simulink model "Chen2003_ExtendedEMF"  (R2024b)
settings: Solver=FixedStepDiscrete  StartTime=0.0  StopTime=.52  FixedStep=Ts  RelTol=1e-3
model workspace (MAT data in the model file):
  Bobs = 850
  ID0 = -2
  IQ0 = 2
  KiPLL = 5600
  KpPLL = 150
  Ld = 0.00159999995958
  Lq = 0.00310000008903
  Omega0 = 280
  PolePairs = 4
  PsiPM = 0.0450000017881
  RecordedSignalNames = {'VAlpha'; 'VBeta'; 'IAlpha'; 'IBeta'; 'ThetaTrue'; 'ID'; 'IQ'; 'Torque'; 'BaselineTheta'; 'BaselineOmega'; 'BaselineEAlpha'; 'BaselineEBeta'; 'EEMFTheta'; 'EEMFOmega'; 'EEMFEAlpha'; 'EEMFEBeta'}
  Rs = 0.20000000298
  ScenarioInput = timeseries
  ScenarioInput.Name = 'unnamed'
  ScenarioInput.DataInfo = tsdata.datametadata
  ScenarioInput.DataInfo.Interpolation = tsdata.interpolation
  ScenarioInput.DataInfo.Interpolation.Fhandle : function handle (value not decoded)
  ScenarioInput.DataInfo.Interpolation.Name = 'linear'
  ScenarioInput.TimeInfo = tsdata.timemetadata
  ScenarioInput.TimeInfo.Length = 10401
  ScenarioInput.TimeInfo.DuplicateTimes = 0
  ScenarioInput.TimeInfo.Time_ = [0 5e-05 0.0001 0.00015 0.0002 0.00025 0.0003 0.00035 0.0004 0.00045 0.0005 0.00055 ... (10401 elements, 10401x1)]
  ScenarioInput.TimeInfo.Initialized = 1
  ScenarioInput.QualityInfo = tsdata.qualmetadata
  ScenarioInput.Data_ = [-7.32373666763 -7.5133357048 -7.70101070404 -7.88671445847 -8.07039928436 -8.25201797485 -8.43152427673 -8.60887241364 -8.78401660919 -8.95691204071 -9.12751483917 -9.29578113556 ... (41604 elements, 10401x4)]
  Theta0 = 0.119999997318
  ThetaPlant = 0.379999995232
  Ts = 5e-05
  Vdc = 60
settings Model: Creator=lxy  LastModifiedBy=lxy

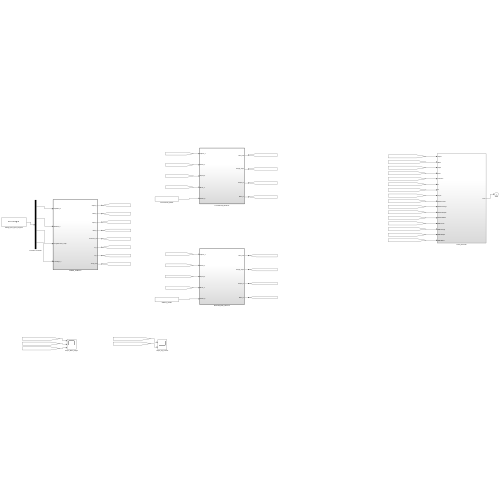
[thumbnail: Simulink's stored preview of the top-level diagram]
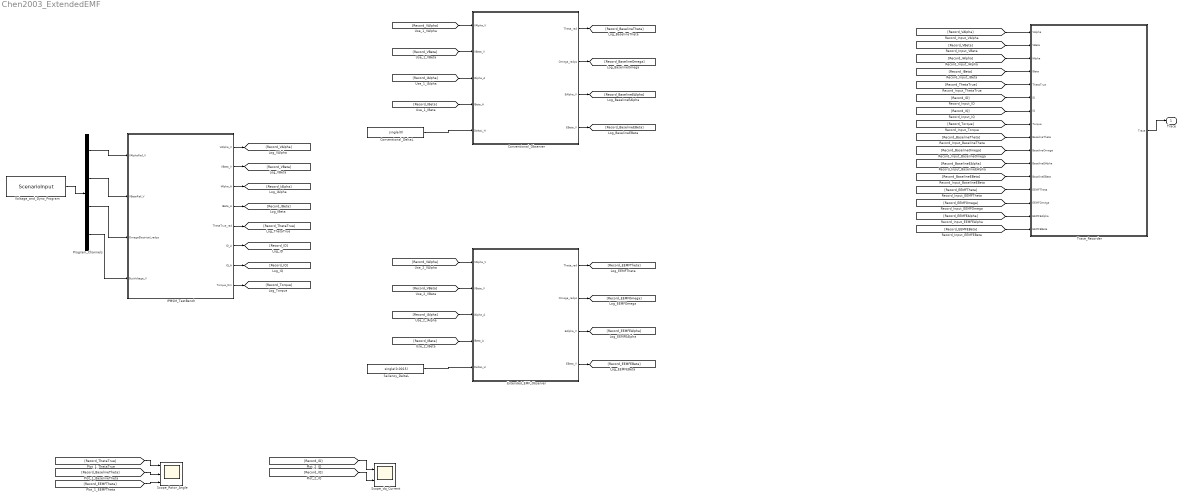
== system Chen2003_ExtendedEMF ==
  Conventional_DeltaL : Constant  Value=single(0)
  Conventional_Observer : Subsystem  TreatAsAtomicUnit=on
  Extended_EMF_Observer : Subsystem  TreatAsAtomicUnit=on
  IPMSM_TestBench : Subsystem  TreatAsAtomicUnit=on
  Program_Channels : Demux
  Saliency_DeltaL : Constant  Value=single(0.0015)
  Scope_Rotor_Angle : Scope  NumInputPorts=3
  Scope_dq_Current : Scope  NumInputPorts=2
  Trace_Recorder : Subsystem
  Voltage_and_Dyno_Program : FromWorkspace  VariableName=ScenarioInput  SampleTime=Ts  Interpolate=off  OutputAfterFinalValue=Holding final value
  Trace : Outport
  wires:
  Program_Channels/4 -> IPMSM_TestBench/4(BusVoltage_V)
  Program_Channels/2 -> IPMSM_TestBench/2(VBetaRef_V)
  Program_Channels/1 -> IPMSM_TestBench/1(VAlphaRef_V)
  Program_Channels/3 -> IPMSM_TestBench/3(OmegaElectrical_radps)
  Voltage_and_Dyno_Program/1 -> Program_Channels/1
  Saliency_DeltaL/1 -> Extended_EMF_Observer/5(DeltaL_H)
  Conventional_DeltaL/1 -> Conventional_Observer/5(DeltaL_H)
  [Record_EEMFEBeta] -> Trace_Recorder/16(EEMFEBeta)
  [Record_EEMFEAlpha] -> Trace_Recorder/15(EEMFEAlpha)
  [Record_EEMFOmega] -> Trace_Recorder/14(EEMFOmega)
  [Record_EEMFTheta] -> Trace_Recorder/13(EEMFTheta)
  [Record_BaselineEBeta] -> Trace_Recorder/12(BaselineEBeta)
  [Record_BaselineEAlpha] -> Trace_Recorder/11(BaselineEAlpha)
  [Record_BaselineOmega] -> Trace_Recorder/10(BaselineOmega)
  [Record_BaselineTheta] -> Trace_Recorder/9(BaselineTheta)
  [Record_Torque] -> Trace_Recorder/8(Torque)
  [Record_IQ] -> Trace_Recorder/7(IQ)
  [Record_ID] -> Trace_Recorder/6(ID)
  [Record_ThetaTrue] -> Trace_Recorder/5(ThetaTrue)
  [Record_IBeta] -> Trace_Recorder/4(IBeta)
  [Record_IAlpha] -> Trace_Recorder/3(IAlpha)
  [Record_VBeta] -> Trace_Recorder/2(VBeta)
  [Record_VAlpha] -> Trace_Recorder/1(VAlpha)
  Trace_Recorder/1(Trace) -> Trace/1
  Extended_EMF_Observer/4(EBeta_V) -> [Record_EEMFEBeta]
  Extended_EMF_Observer/3(EAlpha_V) -> [Record_EEMFEAlpha]
  Extended_EMF_Observer/2(Omega_radps) -> [Record_EEMFOmega]
  Conventional_Observer/4(EBeta_V) -> [Record_BaselineEBeta]
  Conventional_Observer/3(EAlpha_V) -> [Record_BaselineEAlpha]
  Conventional_Observer/2(Omega_radps) -> [Record_BaselineOmega]
  IPMSM_TestBench/8(Torque_Nm) -> [Record_Torque]
  Extended_EMF_Observer/1(Theta_rad) -> [Record_EEMFTheta]
  Conventional_Observer/1(Theta_rad) -> [Record_BaselineTheta]
  IPMSM_TestBench/5(ThetaTrue_rad) -> [Record_ThetaTrue]
  IPMSM_TestBench/2(VBeta_V) -> [Record_VBeta]
  IPMSM_TestBench/1(VAlpha_V) -> [Record_VAlpha]
  IPMSM_TestBench/3(IAlpha_A) -> [Record_IAlpha]
  IPMSM_TestBench/4(IBeta_A) -> [Record_IBeta]
  IPMSM_TestBench/6(ID_A) -> [Record_ID]
  IPMSM_TestBench/7(IQ_A) -> [Record_IQ]
  [Record_IBeta] -> Extended_EMF_Observer/4(IBeta_A)
  [Record_IAlpha] -> Extended_EMF_Observer/3(IAlpha_A)
  [Record_VBeta] -> Extended_EMF_Observer/2(VBeta_V)
  [Record_VAlpha] -> Extended_EMF_Observer/1(VAlpha_V)
  [Record_IBeta] -> Conventional_Observer/4(IBeta_A)
  [Record_IAlpha] -> Conventional_Observer/3(IAlpha_A)
  [Record_VBeta] -> Conventional_Observer/2(VBeta_V)
  [Record_VAlpha] -> Conventional_Observer/1(VAlpha_V)
  [Record_IQ] -> Scope_dq_Current/2
  [Record_ID] -> Scope_dq_Current/1
  [Record_EEMFTheta] -> Scope_Rotor_Angle/3
  [Record_BaselineTheta] -> Scope_Rotor_Angle/2
  [Record_ThetaTrue] -> Scope_Rotor_Angle/1

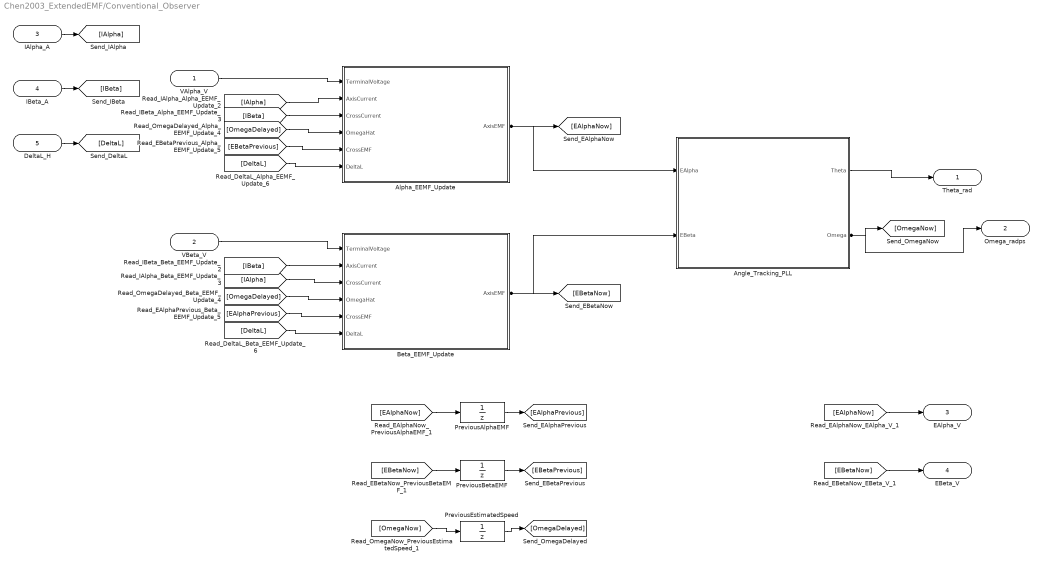
== system Chen2003_ExtendedEMF/Conventional_Observer ==
  VAlpha_V : Inport  OutDataTypeStr=single  SampleTime=Ts
  VBeta_V : Inport  Port=2  OutDataTypeStr=single  SampleTime=Ts
  IAlpha_A : Inport  Port=3  OutDataTypeStr=single  SampleTime=Ts
  IBeta_A : Inport  Port=4  OutDataTypeStr=single  SampleTime=Ts
  DeltaL_H : Inport  Port=5  OutDataTypeStr=single  SampleTime=Ts
  Alpha_EEMF_Update : Subsystem
  Angle_Tracking_PLL : Subsystem
  Beta_EEMF_Update : Subsystem
  PreviousAlphaEMF : UnitDelay  SampleTime=Ts  HasFrameUpgradeWarning=on
  PreviousBetaEMF : UnitDelay  SampleTime=Ts  HasFrameUpgradeWarning=on
  PreviousEstimatedSpeed : UnitDelay  InitialCondition=Omega0  SampleTime=Ts  HasFrameUpgradeWarning=on
  Theta_rad : Outport
  Omega_radps : Outport  Port=2
  EAlpha_V : Outport  Port=3
  EBeta_V : Outport  Port=4
  wires:
  [OmegaDelayed] -> Beta_EEMF_Update/4(OmegaHat)
  [OmegaDelayed] -> Alpha_EEMF_Update/4(OmegaHat)
  PreviousEstimatedSpeed/1 -> [OmegaDelayed]
  [OmegaNow] -> PreviousEstimatedSpeed/1
  [EBetaPrevious] -> Alpha_EEMF_Update/5(CrossEMF)
  PreviousBetaEMF/1 -> [EBetaPrevious]
  [EBetaNow] -> EBeta_V/1
  [EBetaNow] -> PreviousBetaEMF/1
  [EAlphaPrevious] -> Beta_EEMF_Update/5(CrossEMF)
  PreviousAlphaEMF/1 -> [EAlphaPrevious]
  [EAlphaNow] -> EAlpha_V/1
  [EAlphaNow] -> PreviousAlphaEMF/1
  [DeltaL] -> Beta_EEMF_Update/6(DeltaL)
  [DeltaL] -> Alpha_EEMF_Update/6(DeltaL)
  DeltaL_H/1 -> [DeltaL]
  [IBeta] -> Beta_EEMF_Update/2(AxisCurrent)
  [IBeta] -> Alpha_EEMF_Update/3(CrossCurrent)
  IBeta_A/1 -> [IBeta]
  [IAlpha] -> Beta_EEMF_Update/3(CrossCurrent)
  [IAlpha] -> Alpha_EEMF_Update/2(AxisCurrent)
  IAlpha_A/1 -> [IAlpha]
  Angle_Tracking_PLL/2(Omega) -> Omega_radps/1, [OmegaNow]
  Angle_Tracking_PLL/1(Theta) -> Theta_rad/1
  VBeta_V/1 -> Beta_EEMF_Update/1(TerminalVoltage)
  VAlpha_V/1 -> Alpha_EEMF_Update/1(TerminalVoltage)
  Beta_EEMF_Update/1(AxisEMF) -> [EBetaNow], Angle_Tracking_PLL/2(EBeta)
  Alpha_EEMF_Update/1(AxisEMF) -> [EAlphaNow], Angle_Tracking_PLL/1(EAlpha)

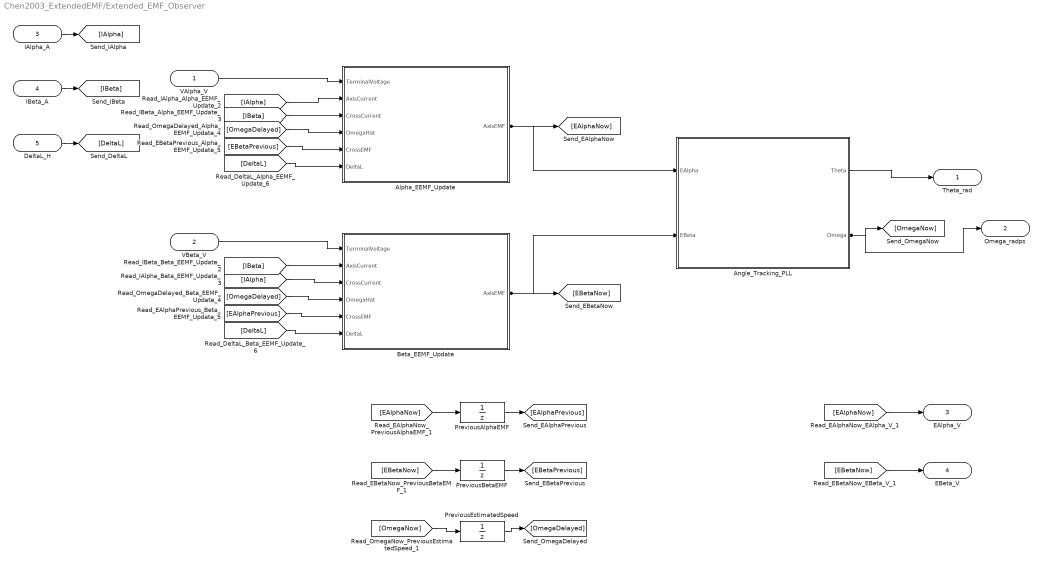
== system Chen2003_ExtendedEMF/Extended_EMF_Observer ==
  VAlpha_V : Inport  OutDataTypeStr=single  SampleTime=Ts
  VBeta_V : Inport  Port=2  OutDataTypeStr=single  SampleTime=Ts
  IAlpha_A : Inport  Port=3  OutDataTypeStr=single  SampleTime=Ts
  IBeta_A : Inport  Port=4  OutDataTypeStr=single  SampleTime=Ts
  DeltaL_H : Inport  Port=5  OutDataTypeStr=single  SampleTime=Ts
  Alpha_EEMF_Update : Subsystem
  Angle_Tracking_PLL : Subsystem
  Beta_EEMF_Update : Subsystem
  PreviousAlphaEMF : UnitDelay  SampleTime=Ts  HasFrameUpgradeWarning=on
  PreviousBetaEMF : UnitDelay  SampleTime=Ts  HasFrameUpgradeWarning=on
  PreviousEstimatedSpeed : UnitDelay  InitialCondition=Omega0  SampleTime=Ts  HasFrameUpgradeWarning=on
  Theta_rad : Outport
  Omega_radps : Outport  Port=2
  EAlpha_V : Outport  Port=3
  EBeta_V : Outport  Port=4
  wires:
  [OmegaDelayed] -> Beta_EEMF_Update/4(OmegaHat)
  [OmegaDelayed] -> Alpha_EEMF_Update/4(OmegaHat)
  PreviousEstimatedSpeed/1 -> [OmegaDelayed]
  [OmegaNow] -> PreviousEstimatedSpeed/1
  [EBetaPrevious] -> Alpha_EEMF_Update/5(CrossEMF)
  PreviousBetaEMF/1 -> [EBetaPrevious]
  [EBetaNow] -> EBeta_V/1
  [EBetaNow] -> PreviousBetaEMF/1
  [EAlphaPrevious] -> Beta_EEMF_Update/5(CrossEMF)
  PreviousAlphaEMF/1 -> [EAlphaPrevious]
  [EAlphaNow] -> EAlpha_V/1
  [EAlphaNow] -> PreviousAlphaEMF/1
  [DeltaL] -> Beta_EEMF_Update/6(DeltaL)
  [DeltaL] -> Alpha_EEMF_Update/6(DeltaL)
  DeltaL_H/1 -> [DeltaL]
  [IBeta] -> Beta_EEMF_Update/2(AxisCurrent)
  [IBeta] -> Alpha_EEMF_Update/3(CrossCurrent)
  IBeta_A/1 -> [IBeta]
  [IAlpha] -> Beta_EEMF_Update/3(CrossCurrent)
  [IAlpha] -> Alpha_EEMF_Update/2(AxisCurrent)
  IAlpha_A/1 -> [IAlpha]
  Angle_Tracking_PLL/2(Omega) -> Omega_radps/1, [OmegaNow]
  Angle_Tracking_PLL/1(Theta) -> Theta_rad/1
  VBeta_V/1 -> Beta_EEMF_Update/1(TerminalVoltage)
  VAlpha_V/1 -> Alpha_EEMF_Update/1(TerminalVoltage)
  Beta_EEMF_Update/1(AxisEMF) -> [EBetaNow], Angle_Tracking_PLL/2(EBeta)
  Alpha_EEMF_Update/1(AxisEMF) -> [EAlphaNow], Angle_Tracking_PLL/1(EAlpha)

== system Chen2003_ExtendedEMF/IPMSM_TestBench ==
  VAlphaRef_V : Inport  OutDataTypeStr=single  SampleTime=Ts
  VBetaRef_V : Inport  Port=2  OutDataTypeStr=single  SampleTime=Ts
  OmegaElectrical_radps : Inport  Port=3  OutDataTypeStr=single  SampleTime=Ts
  BusVoltage_V : Inport  Port=4  OutDataTypeStr=single  SampleTime=Ts
  Average_SVPWM_Inverter : Subsystem
  IPMSM_dq_Voltage_Dynamics : Subsystem
  VAlpha_V : Outport
  VBeta_V : Outport  Port=2
  IAlpha_A : Outport  Port=3
  IBeta_A : Outport  Port=4
  ThetaTrue_rad : Outport  Port=5
  ID_A : Outport  Port=6
  IQ_A : Outport  Port=7
  Torque_Nm : Outport  Port=8
  wires:
  IPMSM_dq_Voltage_Dynamics/6(Torque) -> Torque_Nm/1
  IPMSM_dq_Voltage_Dynamics/5(IQ) -> IQ_A/1
  IPMSM_dq_Voltage_Dynamics/4(ID) -> ID_A/1
  IPMSM_dq_Voltage_Dynamics/3(Theta) -> ThetaTrue_rad/1
  IPMSM_dq_Voltage_Dynamics/2(IBeta) -> IBeta_A/1
  IPMSM_dq_Voltage_Dynamics/1(IAlpha) -> IAlpha_A/1
  OmegaElectrical_radps/1 -> IPMSM_dq_Voltage_Dynamics/3(Omega)
  Average_SVPWM_Inverter/2(VBeta) -> VBeta_V/1, IPMSM_dq_Voltage_Dynamics/2(VBeta)
  Average_SVPWM_Inverter/1(VAlpha) -> VAlpha_V/1, IPMSM_dq_Voltage_Dynamics/1(VAlpha)
  BusVoltage_V/1 -> Average_SVPWM_Inverter/3(BusVoltage)
  VBetaRef_V/1 -> Average_SVPWM_Inverter/2(VBetaRef)
  VAlphaRef_V/1 -> Average_SVPWM_Inverter/1(VAlphaRef)

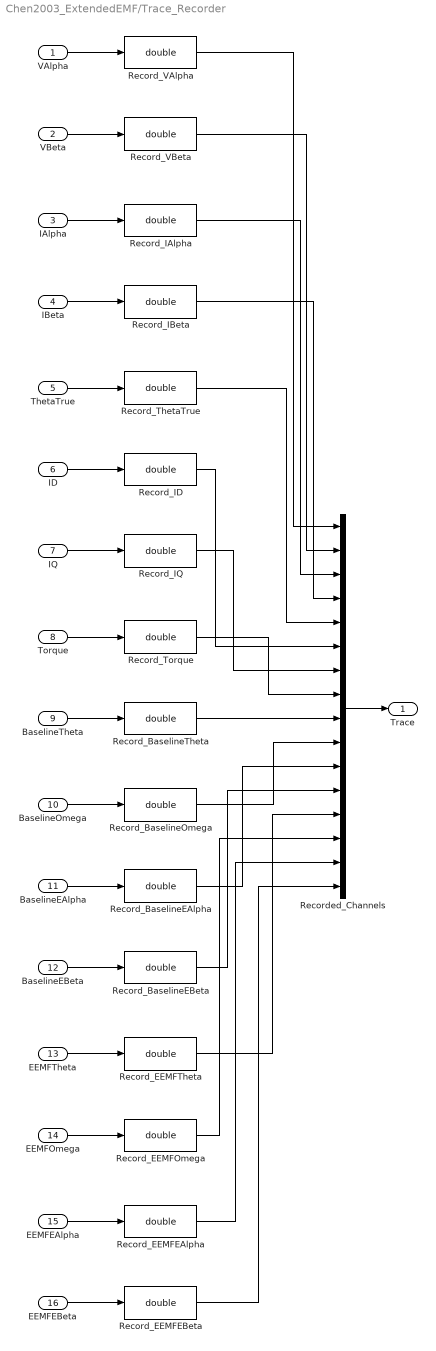
== system Chen2003_ExtendedEMF/Trace_Recorder ==
  VAlpha : Inport
  VBeta : Inport  Port=2
  IAlpha : Inport  Port=3
  IBeta : Inport  Port=4
  ThetaTrue : Inport  Port=5
  ID : Inport  Port=6
  IQ : Inport  Port=7
  Torque : Inport  Port=8
  BaselineTheta : Inport  Port=9
  BaselineOmega : Inport  Port=10
  BaselineEAlpha : Inport  Port=11
  BaselineEBeta : Inport  Port=12
  EEMFTheta : Inport  Port=13
  EEMFOmega : Inport  Port=14
  EEMFEAlpha : Inport  Port=15
  EEMFEBeta : Inport  Port=16
  Record_BaselineEAlpha : DataTypeConversion  OutDataTypeStr=double  SaturateOnIntegerOverflow=off  RndMeth=Floor
  Record_BaselineEBeta : DataTypeConversion  OutDataTypeStr=double  SaturateOnIntegerOverflow=off  RndMeth=Floor
  Record_BaselineOmega : DataTypeConversion  OutDataTypeStr=double  SaturateOnIntegerOverflow=off  RndMeth=Floor
  Record_BaselineTheta : DataTypeConversion  OutDataTypeStr=double  SaturateOnIntegerOverflow=off  RndMeth=Floor
  Record_EEMFEAlpha : DataTypeConversion  OutDataTypeStr=double  SaturateOnIntegerOverflow=off  RndMeth=Floor
  Record_EEMFEBeta : DataTypeConversion  OutDataTypeStr=double  SaturateOnIntegerOverflow=off  RndMeth=Floor
  Record_EEMFOmega : DataTypeConversion  OutDataTypeStr=double  SaturateOnIntegerOverflow=off  RndMeth=Floor
  Record_EEMFTheta : DataTypeConversion  OutDataTypeStr=double  SaturateOnIntegerOverflow=off  RndMeth=Floor
  Record_IAlpha : DataTypeConversion  OutDataTypeStr=double  SaturateOnIntegerOverflow=off  RndMeth=Floor
  Record_IBeta : DataTypeConversion  OutDataTypeStr=double  SaturateOnIntegerOverflow=off  RndMeth=Floor
  Record_ID : DataTypeConversion  OutDataTypeStr=double  SaturateOnIntegerOverflow=off  RndMeth=Floor
  Record_IQ : DataTypeConversion  OutDataTypeStr=double  SaturateOnIntegerOverflow=off  RndMeth=Floor
  Record_ThetaTrue : DataTypeConversion  OutDataTypeStr=double  SaturateOnIntegerOverflow=off  RndMeth=Floor
  Record_Torque : DataTypeConversion  OutDataTypeStr=double  SaturateOnIntegerOverflow=off  RndMeth=Floor
  Record_VAlpha : DataTypeConversion  OutDataTypeStr=double  SaturateOnIntegerOverflow=off  RndMeth=Floor
  Record_VBeta : DataTypeConversion  OutDataTypeStr=double  SaturateOnIntegerOverflow=off  RndMeth=Floor
  Recorded_Channels : Mux  Inputs=16
  Trace : Outport
  wires:
  Recorded_Channels/1 -> Trace/1
  Record_EEMFEBeta/1 -> Recorded_Channels/16
  EEMFEBeta/1 -> Record_EEMFEBeta/1
  Record_EEMFEAlpha/1 -> Recorded_Channels/15
  EEMFEAlpha/1 -> Record_EEMFEAlpha/1
  Record_EEMFOmega/1 -> Recorded_Channels/14
  EEMFOmega/1 -> Record_EEMFOmega/1
  Record_EEMFTheta/1 -> Recorded_Channels/13
  EEMFTheta/1 -> Record_EEMFTheta/1
  Record_BaselineEBeta/1 -> Recorded_Channels/12
  BaselineEBeta/1 -> Record_BaselineEBeta/1
  Record_BaselineEAlpha/1 -> Recorded_Channels/11
  BaselineEAlpha/1 -> Record_BaselineEAlpha/1
  Record_BaselineOmega/1 -> Recorded_Channels/10
  BaselineOmega/1 -> Record_BaselineOmega/1
  Record_BaselineTheta/1 -> Recorded_Channels/9
  BaselineTheta/1 -> Record_BaselineTheta/1
  Record_Torque/1 -> Recorded_Channels/8
  Torque/1 -> Record_Torque/1
  Record_IQ/1 -> Recorded_Channels/7
  IQ/1 -> Record_IQ/1
  Record_ID/1 -> Recorded_Channels/6
  ID/1 -> Record_ID/1
  Record_ThetaTrue/1 -> Recorded_Channels/5
  ThetaTrue/1 -> Record_ThetaTrue/1
  Record_IBeta/1 -> Recorded_Channels/4
  IBeta/1 -> Record_IBeta/1
  Record_IAlpha/1 -> Recorded_Channels/3
  IAlpha/1 -> Record_IAlpha/1
  Record_VBeta/1 -> Recorded_Channels/2
  VBeta/1 -> Record_VBeta/1
  Record_VAlpha/1 -> Recorded_Channels/1
  VAlpha/1 -> Record_VAlpha/1

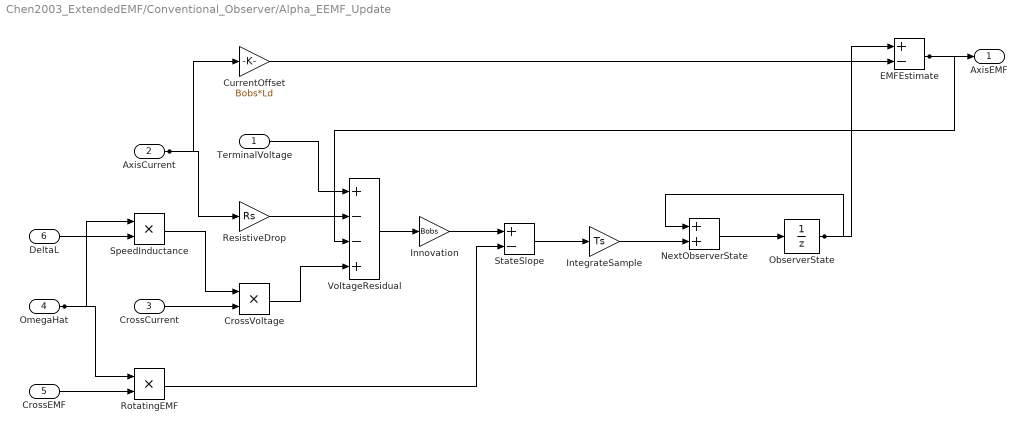
== system Chen2003_ExtendedEMF/Conventional_Observer/Alpha_EEMF_Update ==
  TerminalVoltage : Inport
  AxisCurrent : Inport  Port=2
  CrossCurrent : Inport  Port=3
  OmegaHat : Inport  Port=4
  CrossEMF : Inport  Port=5
  DeltaL : Inport  Port=6
  CrossVoltage : Product  Inputs=**
  CurrentOffset : Gain  Gain=Bobs*Ld
  EMFEstimate : Sum  Inputs=+-
  Innovation : Gain  Gain=Bobs
  IntegrateSample : Gain  Gain=Ts
  NextObserverState : Sum
  ObserverState : UnitDelay  SampleTime=Ts  HasFrameUpgradeWarning=on
  ResistiveDrop : Gain  Gain=Rs
  RotatingEMF : Product  Inputs=**
  SpeedInductance : Product  Inputs=**
  StateSlope : Sum  Inputs=+-
  VoltageResidual : Sum  Inputs=+--+
  AxisEMF : Outport
  wires:
  AxisCurrent/1 -> CurrentOffset/1, ResistiveDrop/1
  ObserverState/1 -> NextObserverState/1, EMFEstimate/1
  CurrentOffset/1 -> EMFEstimate/2
  OmegaHat/1 -> RotatingEMF/1, SpeedInductance/1
  DeltaL/1 -> SpeedInductance/2
  SpeedInductance/1 -> CrossVoltage/1
  CrossCurrent/1 -> CrossVoltage/2
  TerminalVoltage/1 -> VoltageResidual/1
  ResistiveDrop/1 -> VoltageResidual/2
  EMFEstimate/1 -> AxisEMF/1, VoltageResidual/3
  CrossVoltage/1 -> VoltageResidual/4
  VoltageResidual/1 -> Innovation/1
  CrossEMF/1 -> RotatingEMF/2
  Innovation/1 -> StateSlope/1
  RotatingEMF/1 -> StateSlope/2
  StateSlope/1 -> IntegrateSample/1
  IntegrateSample/1 -> NextObserverState/2
  NextObserverState/1 -> ObserverState/1

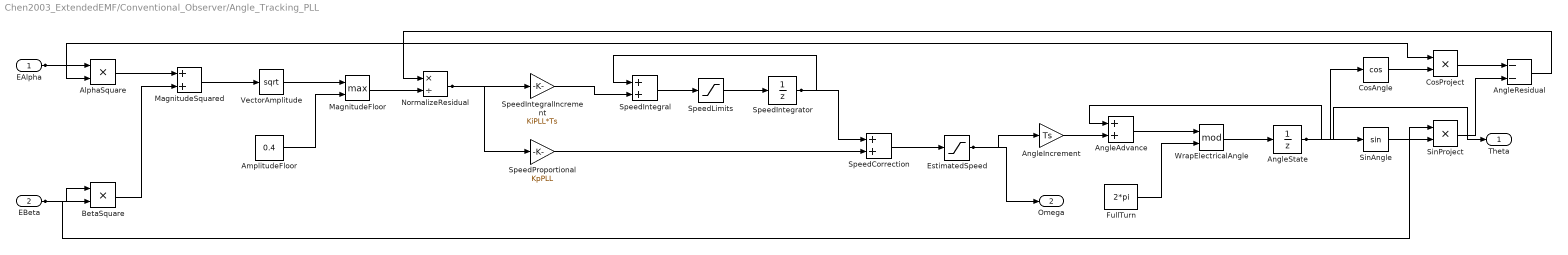
== system Chen2003_ExtendedEMF/Conventional_Observer/Angle_Tracking_PLL ==
  EAlpha : Inport
  EBeta : Inport  Port=2
  AlphaSquare : Product  Inputs=**
  AmplitudeFloor : Constant  Value=0.4  OutDataTypeStr=single
  AngleAdvance : Sum
  AngleIncrement : Gain  Gain=Ts
  AngleResidual : Sum  Inputs=--
  AngleState : UnitDelay  InitialCondition=Theta0  SampleTime=Ts  HasFrameUpgradeWarning=on
  BetaSquare : Product  Inputs=**
  CosAngle : Trigonometry  Operator=cos
  CosProject : Product  Inputs=**
  EstimatedSpeed : Saturate  UpperLimit=900  LowerLimit=40
  FullTurn : Constant  Value=2*pi  OutDataTypeStr=single
  MagnitudeFloor : MinMax  Function=max  Inputs=2
  MagnitudeSquared : Sum
  NormalizeResidual : Product  Inputs=*/
  SinAngle : Trigonometry
  SinProject : Product  Inputs=**
  SpeedCorrection : Sum
  SpeedIntegral : Sum
  SpeedIntegralIncrement : Gain  Gain=KiPLL*Ts
  SpeedIntegrator : UnitDelay  InitialCondition=Omega0  SampleTime=Ts  HasFrameUpgradeWarning=on
  SpeedLimits : Saturate  UpperLimit=900  LowerLimit=40
  SpeedProportional : Gain  Gain=KpPLL
  VectorAmplitude : Sqrt
  WrapElectricalAngle : Math  Operator=mod
  Theta : Outport
  Omega : Outport  Port=2
  wires:
  EAlpha/1 -> CosProject/1, AlphaSquare/1, AlphaSquare/2
  EBeta/1 -> SinProject/1, BetaSquare/1, BetaSquare/2
  AlphaSquare/1 -> MagnitudeSquared/1
  BetaSquare/1 -> MagnitudeSquared/2
  MagnitudeSquared/1 -> VectorAmplitude/1
  VectorAmplitude/1 -> MagnitudeFloor/1
  AmplitudeFloor/1 -> MagnitudeFloor/2
  AngleState/1 -> Theta/1, AngleAdvance/1, SinAngle/1, CosAngle/1
  CosAngle/1 -> CosProject/2
  SinAngle/1 -> SinProject/2
  CosProject/1 -> AngleResidual/1
  SinProject/1 -> AngleResidual/2
  AngleResidual/1 -> NormalizeResidual/1
  MagnitudeFloor/1 -> NormalizeResidual/2
  NormalizeResidual/1 -> SpeedProportional/1, SpeedIntegralIncrement/1
  SpeedIntegrator/1 -> SpeedCorrection/1, SpeedIntegral/1
  SpeedIntegralIncrement/1 -> SpeedIntegral/2
  SpeedIntegral/1 -> SpeedLimits/1
  SpeedLimits/1 -> SpeedIntegrator/1
  SpeedProportional/1 -> SpeedCorrection/2
  SpeedCorrection/1 -> EstimatedSpeed/1
  EstimatedSpeed/1 -> Omega/1, AngleIncrement/1
  AngleIncrement/1 -> AngleAdvance/2
  AngleAdvance/1 -> WrapElectricalAngle/1
  FullTurn/1 -> WrapElectricalAngle/2
  WrapElectricalAngle/1 -> AngleState/1

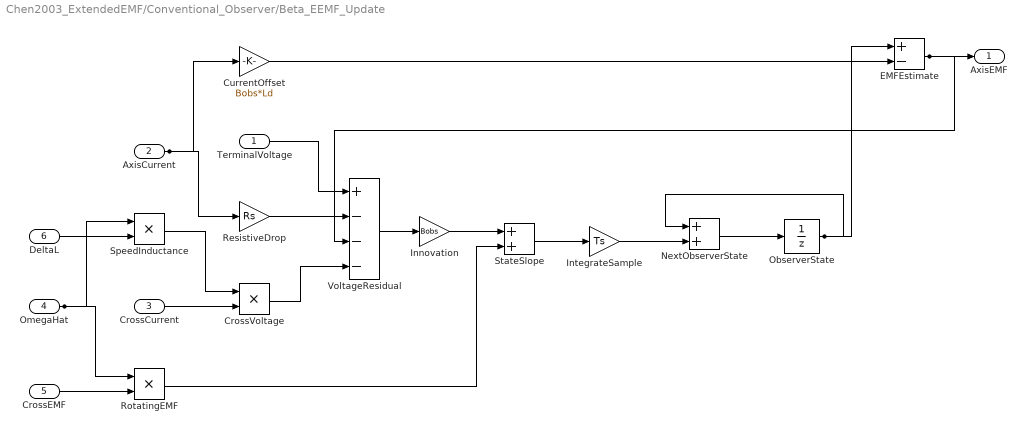
== system Chen2003_ExtendedEMF/Conventional_Observer/Beta_EEMF_Update ==
  TerminalVoltage : Inport
  AxisCurrent : Inport  Port=2
  CrossCurrent : Inport  Port=3
  OmegaHat : Inport  Port=4
  CrossEMF : Inport  Port=5
  DeltaL : Inport  Port=6
  CrossVoltage : Product  Inputs=**
  CurrentOffset : Gain  Gain=Bobs*Ld
  EMFEstimate : Sum  Inputs=+-
  Innovation : Gain  Gain=Bobs
  IntegrateSample : Gain  Gain=Ts
  NextObserverState : Sum
  ObserverState : UnitDelay  SampleTime=Ts  HasFrameUpgradeWarning=on
  ResistiveDrop : Gain  Gain=Rs
  RotatingEMF : Product  Inputs=**
  SpeedInductance : Product  Inputs=**
  StateSlope : Sum
  VoltageResidual : Sum  Inputs=+---
  AxisEMF : Outport
  wires:
  AxisCurrent/1 -> CurrentOffset/1, ResistiveDrop/1
  ObserverState/1 -> NextObserverState/1, EMFEstimate/1
  CurrentOffset/1 -> EMFEstimate/2
  OmegaHat/1 -> RotatingEMF/1, SpeedInductance/1
  DeltaL/1 -> SpeedInductance/2
  SpeedInductance/1 -> CrossVoltage/1
  CrossCurrent/1 -> CrossVoltage/2
  TerminalVoltage/1 -> VoltageResidual/1
  ResistiveDrop/1 -> VoltageResidual/2
  EMFEstimate/1 -> AxisEMF/1, VoltageResidual/3
  CrossVoltage/1 -> VoltageResidual/4
  VoltageResidual/1 -> Innovation/1
  CrossEMF/1 -> RotatingEMF/2
  Innovation/1 -> StateSlope/1
  RotatingEMF/1 -> StateSlope/2
  StateSlope/1 -> IntegrateSample/1
  IntegrateSample/1 -> NextObserverState/2
  NextObserverState/1 -> ObserverState/1

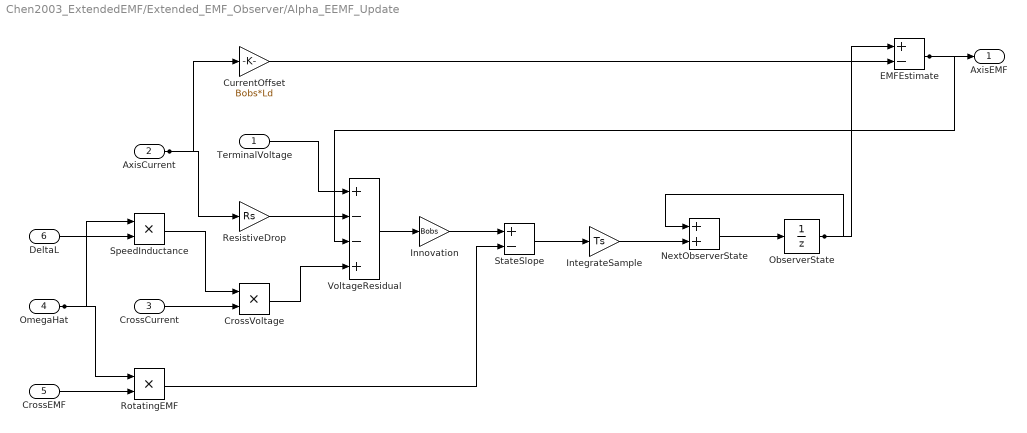
== system Chen2003_ExtendedEMF/Extended_EMF_Observer/Alpha_EEMF_Update ==
  TerminalVoltage : Inport
  AxisCurrent : Inport  Port=2
  CrossCurrent : Inport  Port=3
  OmegaHat : Inport  Port=4
  CrossEMF : Inport  Port=5
  DeltaL : Inport  Port=6
  CrossVoltage : Product  Inputs=**
  CurrentOffset : Gain  Gain=Bobs*Ld
  EMFEstimate : Sum  Inputs=+-
  Innovation : Gain  Gain=Bobs
  IntegrateSample : Gain  Gain=Ts
  NextObserverState : Sum
  ObserverState : UnitDelay  SampleTime=Ts  HasFrameUpgradeWarning=on
  ResistiveDrop : Gain  Gain=Rs
  RotatingEMF : Product  Inputs=**
  SpeedInductance : Product  Inputs=**
  StateSlope : Sum  Inputs=+-
  VoltageResidual : Sum  Inputs=+--+
  AxisEMF : Outport
  wires:
  AxisCurrent/1 -> CurrentOffset/1, ResistiveDrop/1
  ObserverState/1 -> NextObserverState/1, EMFEstimate/1
  CurrentOffset/1 -> EMFEstimate/2
  OmegaHat/1 -> RotatingEMF/1, SpeedInductance/1
  DeltaL/1 -> SpeedInductance/2
  SpeedInductance/1 -> CrossVoltage/1
  CrossCurrent/1 -> CrossVoltage/2
  TerminalVoltage/1 -> VoltageResidual/1
  ResistiveDrop/1 -> VoltageResidual/2
  EMFEstimate/1 -> AxisEMF/1, VoltageResidual/3
  CrossVoltage/1 -> VoltageResidual/4
  VoltageResidual/1 -> Innovation/1
  CrossEMF/1 -> RotatingEMF/2
  Innovation/1 -> StateSlope/1
  RotatingEMF/1 -> StateSlope/2
  StateSlope/1 -> IntegrateSample/1
  IntegrateSample/1 -> NextObserverState/2
  NextObserverState/1 -> ObserverState/1

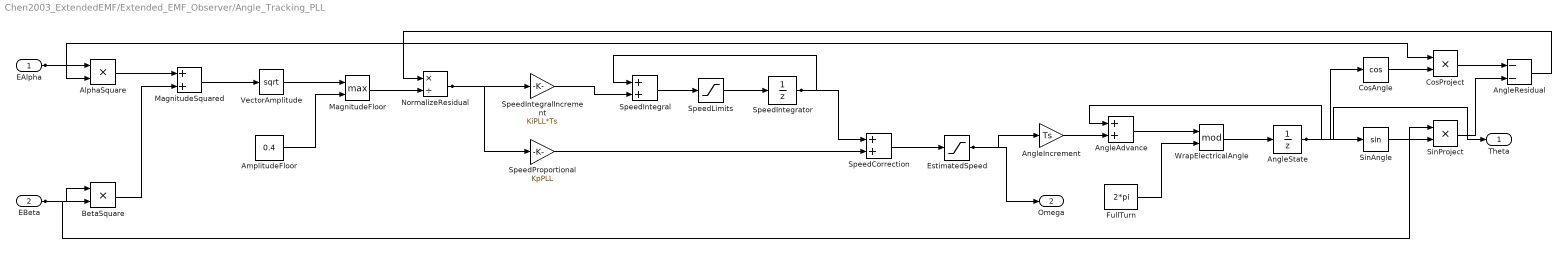
== system Chen2003_ExtendedEMF/Extended_EMF_Observer/Angle_Tracking_PLL ==
  EAlpha : Inport
  EBeta : Inport  Port=2
  AlphaSquare : Product  Inputs=**
  AmplitudeFloor : Constant  Value=0.4  OutDataTypeStr=single
  AngleAdvance : Sum
  AngleIncrement : Gain  Gain=Ts
  AngleResidual : Sum  Inputs=--
  AngleState : UnitDelay  InitialCondition=Theta0  SampleTime=Ts  HasFrameUpgradeWarning=on
  BetaSquare : Product  Inputs=**
  CosAngle : Trigonometry  Operator=cos
  CosProject : Product  Inputs=**
  EstimatedSpeed : Saturate  UpperLimit=900  LowerLimit=40
  FullTurn : Constant  Value=2*pi  OutDataTypeStr=single
  MagnitudeFloor : MinMax  Function=max  Inputs=2
  MagnitudeSquared : Sum
  NormalizeResidual : Product  Inputs=*/
  SinAngle : Trigonometry
  SinProject : Product  Inputs=**
  SpeedCorrection : Sum
  SpeedIntegral : Sum
  SpeedIntegralIncrement : Gain  Gain=KiPLL*Ts
  SpeedIntegrator : UnitDelay  InitialCondition=Omega0  SampleTime=Ts  HasFrameUpgradeWarning=on
  SpeedLimits : Saturate  UpperLimit=900  LowerLimit=40
  SpeedProportional : Gain  Gain=KpPLL
  VectorAmplitude : Sqrt
  WrapElectricalAngle : Math  Operator=mod
  Theta : Outport
  Omega : Outport  Port=2
  wires:
  EAlpha/1 -> CosProject/1, AlphaSquare/1, AlphaSquare/2
  EBeta/1 -> SinProject/1, BetaSquare/1, BetaSquare/2
  AlphaSquare/1 -> MagnitudeSquared/1
  BetaSquare/1 -> MagnitudeSquared/2
  MagnitudeSquared/1 -> VectorAmplitude/1
  VectorAmplitude/1 -> MagnitudeFloor/1
  AmplitudeFloor/1 -> MagnitudeFloor/2
  AngleState/1 -> Theta/1, AngleAdvance/1, SinAngle/1, CosAngle/1
  CosAngle/1 -> CosProject/2
  SinAngle/1 -> SinProject/2
  CosProject/1 -> AngleResidual/1
  SinProject/1 -> AngleResidual/2
  AngleResidual/1 -> NormalizeResidual/1
  MagnitudeFloor/1 -> NormalizeResidual/2
  NormalizeResidual/1 -> SpeedProportional/1, SpeedIntegralIncrement/1
  SpeedIntegrator/1 -> SpeedCorrection/1, SpeedIntegral/1
  SpeedIntegralIncrement/1 -> SpeedIntegral/2
  SpeedIntegral/1 -> SpeedLimits/1
  SpeedLimits/1 -> SpeedIntegrator/1
  SpeedProportional/1 -> SpeedCorrection/2
  SpeedCorrection/1 -> EstimatedSpeed/1
  EstimatedSpeed/1 -> Omega/1, AngleIncrement/1
  AngleIncrement/1 -> AngleAdvance/2
  AngleAdvance/1 -> WrapElectricalAngle/1
  FullTurn/1 -> WrapElectricalAngle/2
  WrapElectricalAngle/1 -> AngleState/1

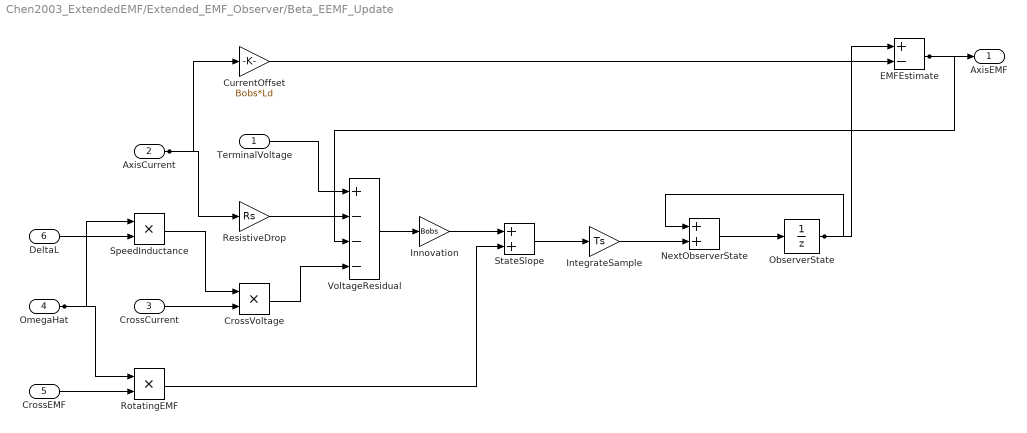
== system Chen2003_ExtendedEMF/Extended_EMF_Observer/Beta_EEMF_Update ==
  TerminalVoltage : Inport
  AxisCurrent : Inport  Port=2
  CrossCurrent : Inport  Port=3
  OmegaHat : Inport  Port=4
  CrossEMF : Inport  Port=5
  DeltaL : Inport  Port=6
  CrossVoltage : Product  Inputs=**
  CurrentOffset : Gain  Gain=Bobs*Ld
  EMFEstimate : Sum  Inputs=+-
  Innovation : Gain  Gain=Bobs
  IntegrateSample : Gain  Gain=Ts
  NextObserverState : Sum
  ObserverState : UnitDelay  SampleTime=Ts  HasFrameUpgradeWarning=on
  ResistiveDrop : Gain  Gain=Rs
  RotatingEMF : Product  Inputs=**
  SpeedInductance : Product  Inputs=**
  StateSlope : Sum
  VoltageResidual : Sum  Inputs=+---
  AxisEMF : Outport
  wires:
  AxisCurrent/1 -> CurrentOffset/1, ResistiveDrop/1
  ObserverState/1 -> NextObserverState/1, EMFEstimate/1
  CurrentOffset/1 -> EMFEstimate/2
  OmegaHat/1 -> RotatingEMF/1, SpeedInductance/1
  DeltaL/1 -> SpeedInductance/2
  SpeedInductance/1 -> CrossVoltage/1
  CrossCurrent/1 -> CrossVoltage/2
  TerminalVoltage/1 -> VoltageResidual/1
  ResistiveDrop/1 -> VoltageResidual/2
  EMFEstimate/1 -> AxisEMF/1, VoltageResidual/3
  CrossVoltage/1 -> VoltageResidual/4
  VoltageResidual/1 -> Innovation/1
  CrossEMF/1 -> RotatingEMF/2
  Innovation/1 -> StateSlope/1
  RotatingEMF/1 -> StateSlope/2
  StateSlope/1 -> IntegrateSample/1
  IntegrateSample/1 -> NextObserverState/2
  NextObserverState/1 -> ObserverState/1

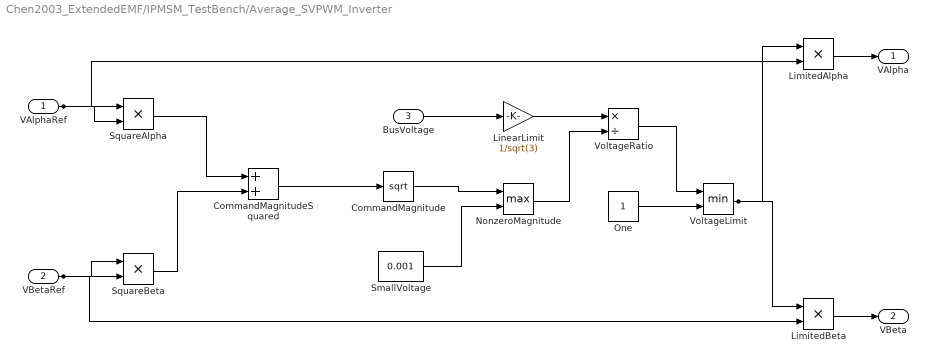
== system Chen2003_ExtendedEMF/IPMSM_TestBench/Average_SVPWM_Inverter ==
  VAlphaRef : Inport
  VBetaRef : Inport  Port=2
  BusVoltage : Inport  Port=3
  CommandMagnitude : Sqrt
  CommandMagnitudeSquared : Sum
  LimitedAlpha : Product  Inputs=**
  LimitedBeta : Product  Inputs=**
  LinearLimit : Gain  Gain=1/sqrt(3)
  NonzeroMagnitude : MinMax  Function=max  Inputs=2
  One : Constant  OutDataTypeStr=single
  SmallVoltage : Constant  Value=0.001  OutDataTypeStr=single
  SquareAlpha : Product  Inputs=**
  SquareBeta : Product  Inputs=**
  VoltageLimit : MinMax  Inputs=2
  VoltageRatio : Product  Inputs=*/
  VAlpha : Outport
  VBeta : Outport  Port=2
  wires:
  VAlphaRef/1 -> LimitedAlpha/2, SquareAlpha/2, SquareAlpha/1
  VBetaRef/1 -> LimitedBeta/2, SquareBeta/2, SquareBeta/1
  SquareAlpha/1 -> CommandMagnitudeSquared/1
  SquareBeta/1 -> CommandMagnitudeSquared/2
  CommandMagnitudeSquared/1 -> CommandMagnitude/1
  CommandMagnitude/1 -> NonzeroMagnitude/1
  SmallVoltage/1 -> NonzeroMagnitude/2
  BusVoltage/1 -> LinearLimit/1
  LinearLimit/1 -> VoltageRatio/1
  NonzeroMagnitude/1 -> VoltageRatio/2
  VoltageRatio/1 -> VoltageLimit/1
  One/1 -> VoltageLimit/2
  VoltageLimit/1 -> LimitedBeta/1, LimitedAlpha/1
  LimitedAlpha/1 -> VAlpha/1
  LimitedBeta/1 -> VBeta/1

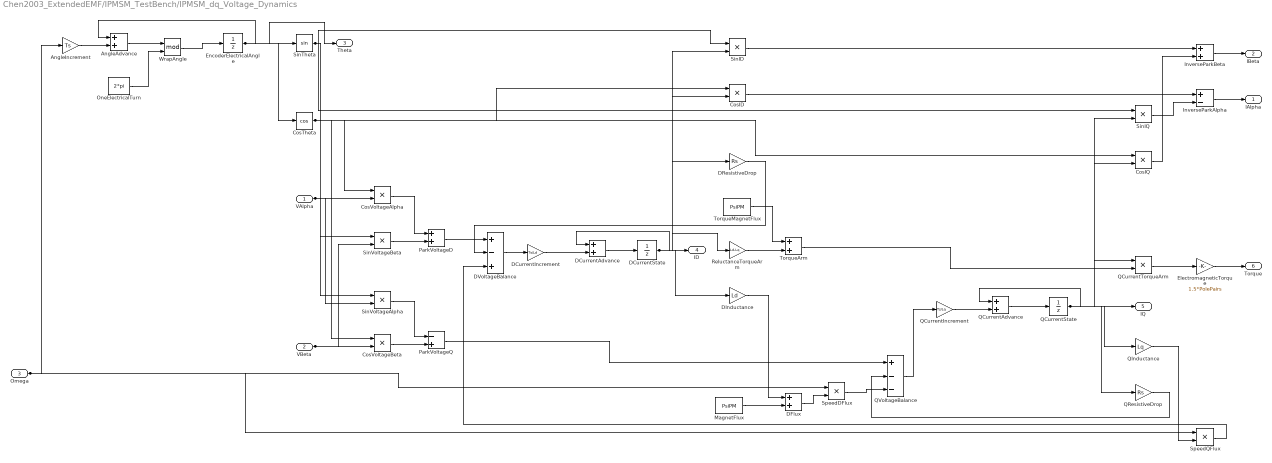
== system Chen2003_ExtendedEMF/IPMSM_TestBench/IPMSM_dq_Voltage_Dynamics ==
  VAlpha : Inport
  VBeta : Inport  Port=2
  Omega : Inport  Port=3
  AngleAdvance : Sum
  AngleIncrement : Gain  Gain=Ts
  CosID : Product  Inputs=**
  CosIQ : Product  Inputs=**
  CosTheta : Trigonometry  Operator=cos
  CosVoltageAlpha : Product  Inputs=**
  CosVoltageBeta : Product  Inputs=**
  DCurrentAdvance : Sum
  DCurrentIncrement : Gain  Gain=Ts/Ld
  DCurrentState : UnitDelay  InitialCondition=ID0  SampleTime=Ts  HasFrameUpgradeWarning=on
  DFlux : Sum
  DInductance : Gain  Gain=Ld
  DResistiveDrop : Gain  Gain=Rs
  DVoltageBalance : Sum  Inputs=+-+
  ElectromagneticTorque : Gain  Gain=1.5*PolePairs
  EncoderElectricalAngle : UnitDelay  InitialCondition=ThetaPlant  SampleTime=Ts  HasFrameUpgradeWarning=on
  InverseParkAlpha : Sum  Inputs=+-
  InverseParkBeta : Sum
  MagnetFlux : Constant  Value=PsiPM  OutDataTypeStr=single
  OneElectricalTurn : Constant  Value=2*pi  OutDataTypeStr=single
  ParkVoltageD : Sum
  ParkVoltageQ : Sum  Inputs=-+
  QCurrentAdvance : Sum
  QCurrentIncrement : Gain  Gain=Ts/Lq
  QCurrentState : UnitDelay  InitialCondition=IQ0  SampleTime=Ts  HasFrameUpgradeWarning=on
  QCurrentTorqueArm : Product  Inputs=**
  QInductance : Gain  Gain=Lq
  QResistiveDrop : Gain  Gain=Rs
  QVoltageBalance : Sum  Inputs=+--
  ReluctanceTorqueArm : Gain  Gain=Ld-Lq
  SinID : Product  Inputs=**
  SinIQ : Product  Inputs=**
  SinTheta : Trigonometry
  SinVoltageAlpha : Product  Inputs=**
  SinVoltageBeta : Product  Inputs=**
  SpeedDFlux : Product  Inputs=**
  SpeedQFlux : Product  Inputs=**
  TorqueArm : Sum
  TorqueMagnetFlux : Constant  Value=PsiPM  OutDataTypeStr=single
  WrapAngle : Math  Operator=mod
  IAlpha : Outport
  IBeta : Outport  Port=2
  Theta : Outport  Port=3
  ID : Outport  Port=4
  IQ : Outport  Port=5
  Torque : Outport  Port=6
  wires:
  Omega/1 -> SpeedDFlux/1, SpeedQFlux/1, AngleIncrement/1
  EncoderElectricalAngle/1 -> Theta/1, AngleAdvance/1, SinTheta/1, CosTheta/1
  AngleIncrement/1 -> AngleAdvance/2
  AngleAdvance/1 -> WrapAngle/1
  OneElectricalTurn/1 -> WrapAngle/2
  WrapAngle/1 -> EncoderElectricalAngle/1
  CosTheta/1 -> CosIQ/1, CosVoltageAlpha/1, CosID/1, CosVoltageBeta/1
  VAlpha/1 -> SinVoltageAlpha/2, CosVoltageAlpha/2
  SinTheta/1 -> SinID/1, SinIQ/1, SinVoltageBeta/1, SinVoltageAlpha/1
  VBeta/1 -> CosVoltageBeta/2, SinVoltageBeta/2
  CosVoltageAlpha/1 -> ParkVoltageD/1
  SinVoltageBeta/1 -> ParkVoltageD/2
  SinVoltageAlpha/1 -> ParkVoltageQ/1
  CosVoltageBeta/1 -> ParkVoltageQ/2
  DCurrentState/1 -> SinID/2, CosID/2, ReluctanceTorqueArm/1, ID/1, DResistiveDrop/1, DCurrentAdvance/1, DInductance/1
  DInductance/1 -> DFlux/1
  MagnetFlux/1 -> DFlux/2
  QCurrentState/1 -> CosIQ/2, SinIQ/2, QResistiveDrop/1, IQ/1, QCurrentAdvance/1, QCurrentTorqueArm/1, QInductance/1
  QInductance/1 -> SpeedQFlux/2
  ParkVoltageD/1 -> DVoltageBalance/1
  DResistiveDrop/1 -> DVoltageBalance/2
  SpeedQFlux/1 -> DVoltageBalance/3
  DFlux/1 -> SpeedDFlux/2
  ParkVoltageQ/1 -> QVoltageBalance/1
  QResistiveDrop/1 -> QVoltageBalance/2
  SpeedDFlux/1 -> QVoltageBalance/3
  DVoltageBalance/1 -> DCurrentIncrement/1
  DCurrentIncrement/1 -> DCurrentAdvance/2
  DCurrentAdvance/1 -> DCurrentState/1
  QVoltageBalance/1 -> QCurrentIncrement/1
  QCurrentIncrement/1 -> QCurrentAdvance/2
  QCurrentAdvance/1 -> QCurrentState/1
  CosID/1 -> InverseParkAlpha/1
  SinIQ/1 -> InverseParkAlpha/2
  SinID/1 -> InverseParkBeta/1
  CosIQ/1 -> InverseParkBeta/2
  TorqueMagnetFlux/1 -> TorqueArm/1
  ReluctanceTorqueArm/1 -> TorqueArm/2
  TorqueArm/1 -> QCurrentTorqueArm/2
  QCurrentTorqueArm/1 -> ElectromagneticTorque/1
  InverseParkAlpha/1 -> IAlpha/1
  InverseParkBeta/1 -> IBeta/1
  ElectromagneticTorque/1 -> Torque/1
